simulink model "TServoSmoothInLoop"  (R2025b)
settings: Solver=ode4  StartTime=0.0  StopTime=inf  FixedStep=0.01  RelTol=1e-3
InitFcn:
  | load("pre-design_data")
libraries: ASEToolBox x11, simulink x1
settings Model: Creator=admin  LastModifiedBy=zqhkd
settings DataIOCC: SaveFinalState=on  SaveOutput=off  InspectSignalLogs=on  SaveTime=off
settings OptimizationCC: EnhancedBackFolding=on  PassReuseOutputArgsAs=Individual arguments  ZeroExternalMemoryAtStartup=off  ZeroInternalMemoryAtStartup=off  OptimizeBlockOrder=speed  DifferentSizesBufferReuse=on  OptimizationCustomize=off  EfficientTunableParamExpr=on
settings DebuggingCC: ParameterTunabilityLossMsg=error
settings HardwareCC: ProdBitPerLong=64.0  ProdHWDeviceType=Intel->x86-64 (Linux 64)
settings SFSimCC: MATLABDynamicMemAlloc=off
settings RTWCC: SystemTargetFile=ert.tlc  TemplateMakefile=ert_default_tmf  RetainRTWFile=on  Toolchain=Microsoft Visual C++ 2022 v17.0 | nmake (64-bit Windows)  GPUComputeCapability=3.5  Description=Embedded Coder
settings CodeAppCC: ForceParamTrailComments=on  IgnoreCustomStorageClasses=off  OperatorAnnotations=on  SimulinkDataObjDesc=on  SFDataObjDesc=on  InsertBlockDesc=on
settings ERTTargetCC: InlinedParameterPlacement=Hierarchical  RTWCAPISignals=on  RTWCAPIParams=on  RTWCAPIStates=on  RTWCAPIRootIO=on  ERTCustomFileTemplate=example_file_process.tlc  DynamicArrayContainerType=coder::array  TargetLangStandard=C99 (ISO)  SupportContinuousTime=on

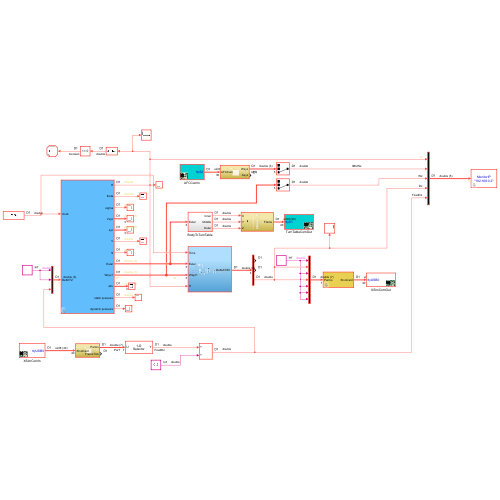
[thumbnail: Simulink's stored preview of the top-level diagram]
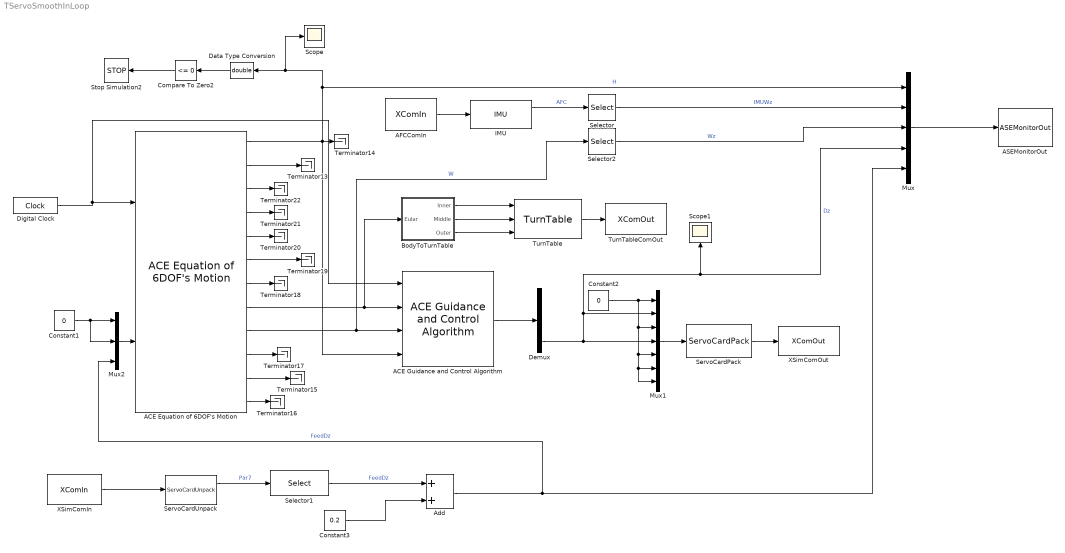
== system TServoSmoothInLoop ==
  ACE Equation of 6DOF's Motion : ASEToolBox/Aerocraft Model/ACE Equation of 6DOF's Motion
      settings: SourceProductName=ASEToolBox
  ACE Guidance and Control Algorithm : ASEToolBox/Aerocraft Model/ACE Guidance and Control Algorithm  SystemSampleTime=-1  VariantActivationTime=update diagram  EmptyChoice=off  PassThrough=off  PassThroughVariantControl=(default)  EmptyChoiceVariantControl=(default)  AllowFlexibleInterface=on  Latency=0  AutoFrameSizeCalculation=off
      settings: SourceProductName=ASEToolBox
  AFCComIn : ASEToolBox/COMModule/XComIn  g_serial_select=ttyS2  g_baudrate=460800  g_parity=None  g_databit=8  g_stopbit=1  g_data_size=6*4+12  g_sample_time=0.01
      settings: SourceProductName=ASEToolBox
  ASEMonitorOut : ASEToolBox/SIMSystemModule/ASEMonitorOut  Tag=ASEMonitorOutTag  g_iVarNum=12  g_iFrameType=10  g_hostIP="\"192.168.0.2\""
      settings: SourceProductName=ASEToolBox
  Add : Sum
  BodyToTurnTable : Subsystem
  Compare To Zero2 : simulink/Logic and Bit Operations/Compare To Zero  relop=<=  OutDataTypeStr=boolean
  Constant1 : Constant  Value=0
  Constant2 : Constant  Value=0
  Constant3 : Constant  Value=0.2
  Data Type Conversion : DataTypeConversion  OutDataTypeStr=double  SaturateOnIntegerOverflow=off  RndMeth=Floor
  Demux : Demux  Outputs=3
  Digital Clock : DigitalClock  SampleTime=0.01
  IMU : ASEToolBox/ACEModule/IMU  SystemSampleTime=-1  VariantActivationTime=update diagram  EmptyChoice=off  PassThrough=off  PassThroughVariantControl=(default)  EmptyChoiceVariantControl=(default)  AllowFlexibleInterface=on  Latency=0  AutoFrameSizeCalculation=off
      settings: SourceProductName=ASEToolBox
  Mux : Mux  Inputs=5
  Mux1 : Mux  Inputs=7
  Mux2 : Mux  Inputs=3
  Scope : Scope
      settings: ActiveDisplayYMinimum=-95.55775  ActiveDisplayYMaximum=860.02971
  Scope1 : Scope
      settings: ActiveDisplayYMinimum=-1.47896  ActiveDisplayYMaximum=4.26221
  Selector : Selector  InputPortWidth=3  IndexOptions=Index vector (dialog)  Indices=3  OutputSizes=1
  Selector1 : Selector  InputPortWidth=7  IndexOptions=Index vector (dialog)  Indices=2  OutputSizes=1
  Selector2 : Selector  InputPortWidth=3  IndexOptions=Index vector (dialog)  Indices=3  OutputSizes=1
  ServoCardPack : ASEToolBox/ACEModule/ServoCardPack  g_FrameType=80  g_SendId=0
      settings: SourceProductName=ASEToolBox
  ServoCardUnpack : ASEToolBox/ACEModule/ServoCardUnpack  SystemSampleTime=-1  VariantActivationTime=update diagram  EmptyChoice=off  PassThrough=off  PassThroughVariantControl=(default)  EmptyChoiceVariantControl=(default)  AllowFlexibleInterface=on  Latency=0  AutoFrameSizeCalculation=off
      settings: SourceProductName=ASEToolBox
  Stop Simulation2 : Stop
  Terminator{13..22} (10 alike) : Terminator
  TurnTable : ASEToolBox/ACEModule/TurnTable  SystemSampleTime=-1  VariantActivationTime=update diagram  EmptyChoice=off  PassThrough=off  PassThroughVariantControl=(default)  EmptyChoiceVariantControl=(default)  AllowFlexibleInterface=on  Latency=0  AutoFrameSizeCalculation=off
      settings: SourceProductName=ASEToolBox
  TurnTableComOut : ASEToolBox/COMModule/XComOut  g_serial_select=ttyS1  g_baudrate=460800  g_parity=None  g_databit=8  g_stopbit=1  g_sample_time=0.01
      settings: SourceProductName=ASEToolBox
  XSimComIn : ASEToolBox/COMModule/XComIn  g_serial_select=ttyUSB0  g_baudrate=460800  g_parity=None  g_databit=8  g_stopbit=1  g_data_size=12+7*4  g_sample_time=0.01
      settings: SourceProductName=ASEToolBox
  XSimComOut : ASEToolBox/COMModule/XComOut  g_serial_select=ttyUSB0  g_baudrate=460800  g_parity=None  g_databit=8  g_stopbit=1  g_sample_time=0.01
      settings: SourceProductName=ASEToolBox
  wires:
  ACE Equation of 6DOF's Motion/11 -> Terminator15/1
  ACE Equation of 6DOF's Motion/3 -> Terminator22/1
  ACE Equation of 6DOF's Motion/7 -> Terminator18/1
  ACE Equation of 6DOF's Motion/8 -> ACE Guidance and Control Algorithm/2, BodyToTurnTable/1(Eular)
  ACE Equation of 6DOF's Motion/2 -> Terminator13/1
  ACE Equation of 6DOF's Motion/12 -> Terminator16/1
  ACE Equation of 6DOF's Motion/1 -> ACE Guidance and Control Algorithm/4, Scope/1, Data Type Conversion/1, Mux/1, Terminator14/1  "H"
  ACE Equation of 6DOF's Motion/4 -> Terminator21/1
  Compare To Zero2/1 -> Stop Simulation2/1
  ACE Equation of 6DOF's Motion/6 -> Terminator19/1
  Digital Clock/1 -> ACE Guidance and Control Algorithm/1, ACE Equation of 6DOF's Motion/1
  ACE Equation of 6DOF's Motion/5 -> Terminator20/1
  ACE Equation of 6DOF's Motion/10 -> Terminator17/1
  Data Type Conversion/1 -> Compare To Zero2/1
  BodyToTurnTable/1(Inner) -> TurnTable/1
  BodyToTurnTable/2(Middle) -> TurnTable/2
  BodyToTurnTable/3(Outer) -> TurnTable/3
  IMU/1 -> Selector/1  "AFC"
  Mux/1 -> ASEMonitorOut/1
  ACE Equation of 6DOF's Motion/9 -> ACE Guidance and Control Algorithm/3, Selector2/1  "W"
  Constant2/1 -> Mux1/7, Mux1/6, Mux1/5, Mux1/3, Mux1/1
  Demux/3 -> Scope1/1, Mux/4, Mux1/2, Mux1/4  "Dz"
  ServoCardUnpack/1 -> Selector1/1  "Par7"
  Selector2/1 -> Mux/3  "Wz"
  Selector/1 -> Mux/2  "IMUWz"
  Mux2/1 -> ACE Equation of 6DOF's Motion/2
  Constant1/1 -> Mux2/2, Mux2/1
  ACE Guidance and Control Algorithm/1 -> Demux/1
  Selector1/1 -> Add/1  "FeedDz"
  Constant3/1 -> Add/2
  XSimComIn/1 -> ServoCardUnpack/1
  ServoCardPack/1 -> XSimComOut/1
  Mux1/1 -> ServoCardPack/1
  AFCComIn/1 -> IMU/1
  TurnTable/1 -> TurnTableComOut/1
  Add/1 -> Mux2/3, Mux/5  "FeedDz"

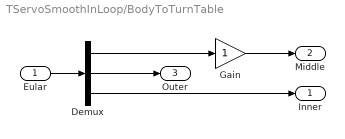
== system TServoSmoothInLoop/BodyToTurnTable ==
  Eular : Inport
  Demux : Demux  Outputs=3
  Gain : Gain
  Inner : Outport
  Middle : Outport  Port=2
  Outer : Outport  Port=3
  wires:
  Demux/1 -> Gain/1
  Eular/1 -> Demux/1
  Gain/1 -> Middle/1
  Demux/3 -> Inner/1
  Demux/2 -> Outer/1
